simulink model "model8_train"  (R2024b)
settings: Solver=VariableStepAuto  StartTime=0.0  StopTime=24  RelTol=1e-3
model workspace (MAT data in the model file):
  agentObj = 67
undefined symbols (not defined in the file): bat_deseado, bat_inicial, difh, dni, e_inicial, ghi, glb, n_inicial, seed_radiation, seed_solar, seed_x, seed_y, seed_z, selection, sun_vector, viento
libraries: rllib x3
settings Model: Creator=danie  LastModifiedBy=Daniel
settings SolverCC: ZeroCrossAlgorithm=Adaptive
settings DebuggingCC: IgnoredZcDiagnostic=none

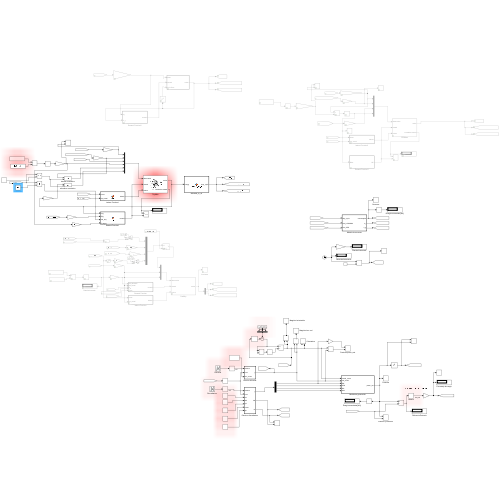
[thumbnail: Simulink's stored preview of the top-level diagram]
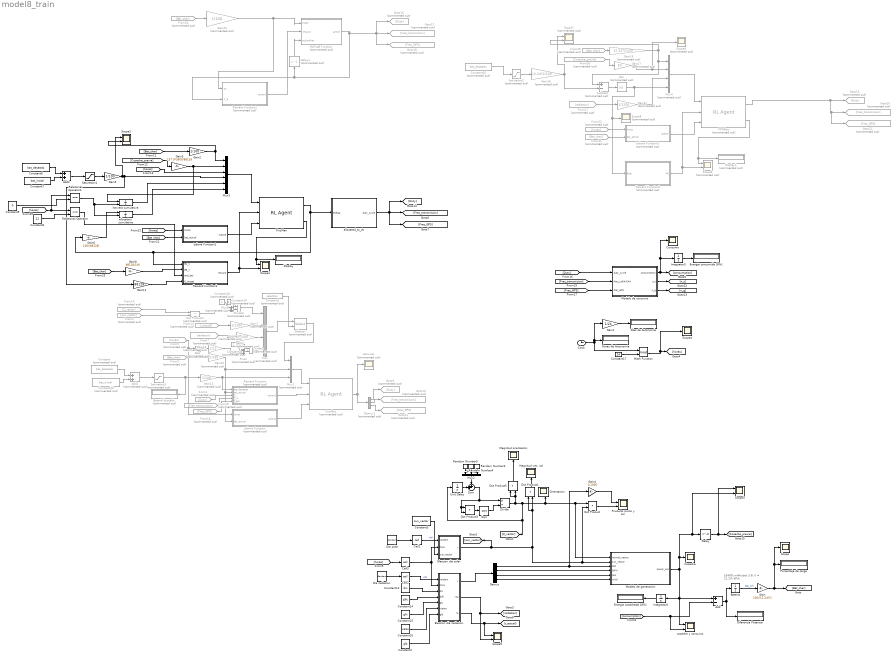
== system model8_train ==
  note: $3400\:mAh\cdot 3.6\:V = 12.24\:Wh$
  Abs : Abs  Commented=on  SaturateOnIntegerOverflow=off
  Acciones : Scope  Commented=on
  Add : Sum  Inputs=+-
  Add1 : Sum  Commented=on
  Add2 : Sum
  Batería : Integrator  InitialCondition=12.24*2*(bat_inicial/100)  LimitOutput=on  UpperSaturationLimit=12.24*2  LowerSaturationLimit=0
  Batería buscado : Display  Commented=on
  Bias : Bias  Commented=on  Bias=-12  SaturateOnIntegerOverflow=off
  Ceil1 : Rounding  Operator=ceil
  Ceil2 : Rounding  Operator=ceil
  Ceil3 : Rounding  Operator=ceil
  Clock : Clock
  Constant : Constant  Commented=on  Value=bat_deseado
  Constant1 : Constant  Commented=on  Value=selection
  Constant10 : Constant  Commented=on  Value=bat_deseado
  Constant13 : Constant  Value=dni
  Constant14 : Constant  Value=difh
  Constant15 : Constant  Value=ghi
  Constant16 : Constant  Value=viento
  Constant17 : Constant  Value=24
  Constant18 : Constant  Commented=on
  Constant19 : Constant  Commented=on  Value=2
  Constant2 : Constant  Value=glb
  Constant20 : Constant  Commented=on  Value=bat_inicial
  Constant3 : Constant  Value=sun_vector
  Constant4 : Constant  Commented=on
  Constant5 : Constant  Commented=on  Value=2
  Constant6 : Constant  Value=bat_deseado
  Constant7 : Constant  Value=bat_inicial
  Constant8 : Constant  Value=22
  Constant9 : Constant  Value=0
  Consumo : Scope
  Cosecha : Scope
  CowBoy : rllib/RL Agent  Commented=on  Agent=agent  ExternalActionAsInput=off  ProvideLastAction=off  ProvideCumRwd=off  TreatAsDirectFeedthrough=on  UseStrictObservationDataTypes=off
  Delay : Delay  DelayLength=0  SampleTime=1
  Delay1 : Delay  Commented=on  DelayLength=1
  Demux : Demux
  Demux1 : Demux  Commented=on  Outputs=3
  Diferencia Potencia : Display
  Display : Display
  Display1 : Display  Commented=on
  Divide : Product  Inputs=*/
  Divide1 : Product  Commented=on  Inputs=/*
  Divide3 : Product  Commented=on  Inputs=/*
  Dot Product{,1,3,5} (4 alike) : DotProduct  OutDataTypeStr=Inherit: Inherit via internal rule
  Dot Product4 : DotProduct  Commented=on  OutDataTypeStr=Inherit: Inherit via internal rule
  Día radiacion : UniformRandomNumber  Minimum=1  Maximum=4383  Seed=seed_radiation  SampleTime=24
  Día solar : UniformRandomNumber  Minimum=1  Maximum=365  Seed=seed_solar  SampleTime=24
  Días de Autonomía : Display
  Eleccion día radiacion : MATLAB Function  TreatAsAtomicUnit=on
  Eleccion día solar : MATLAB Function  TreatAsAtomicUnit=on
  Energia consumida [Wh] : Display
      settings: Decimation=5
  Energia cosechada [Wh] : Display
      settings: Decimation=5
  From1 : From  Commented=on  GotoTag=Duty
  From10 : From  Commented=on  GotoTag=Z_vector
  From14 : From  Commented=on  GotoTag=r_actual
  From18 : From  Commented=on  GotoTag=Frec_GPS
  From19 : From  Commented=on  GotoTag=Frec_transmision
  From2 : From  Commented=on  GotoTag=sun_vector
  From{3,24..25,31} (4 alike) : From  Commented=on  GotoTag=Bat_char
  From26 : From  Commented=on  GotoTag=Cosecha_previa
  From27 : From  Commented=on  GotoTag=radiation
  From32 : From  Commented=on  GotoTag=horas
  From5 : From  Commented=on  GotoTag=horas
  From7 : From  Commented=on  GotoTag=radiation
  Gain : Gain  Gain=100/(12.24*2)
  Gain1 : Gain  Gain=1/24
  Gain10 : Gain  Commented=on  Gain=1/100
  Gain11 : Gain  Gain=88128
  Gain12 : Gain  Commented=on  Gain=1/12
  Gain13 : Gain  Commented=on  Gain=1/100
  Gain15 : Gain  Commented=on  Gain=1/100
  Gain16 : Gain  Commented=on  Gain=12.24*2/100
  Gain17 : Gain  Commented=on  Gain=50
  Gain18 : Gain  Commented=on  Gain=12.24*2/100
  Gain2 : Gain  Gain=1/100
  Gain21 : Gain  Commented=on  Gain=1/1200
  Gain3 : Gain  Gain=157.5*3600/88128
  Gain4 : Gain  Gain=1/1000
  Gain5 : Gain  Gain=1/100
  Gain6 : Gain  Gain=100/(88128)
  Gain7 : Gain  Commented=on  Gain=1/1200
  Gain8 : Gain  Gain=88128/100
  Gain9 : Gain  Commented=on  Gain=1/1200
  Goto10 : Goto  Commented=on  GotoTag=Frec_transmision
  Goto11 : Goto  Commented=on  GotoTag=Frec_GPS
  Goto16 : Goto  Commented=on  GotoTag=Duty
  Goto17 : Goto  Commented=on  GotoTag=Frec_transmision
  Goto18 : Goto  Commented=on  GotoTag=Frec_GPS
  Goto19 : Goto  Commented=on  GotoTag=Duty
  Goto20 : Goto  Commented=on  GotoTag=Frec_transmision
  Goto21 : Goto  Commented=on  GotoTag=Frec_GPS
  Goto9 : Goto  Commented=on  GotoTag=Duty
  Horas de Autonomía : Display
  Integrator3 : Integrator
  Integrator6 : Integrator
  Isdone Function : MATLAB Function  Commented=on  TreatAsAtomicUnit=on
  Isdone Function1 : MATLAB Function  TreatAsAtomicUnit=on
  Isdone Function3 : MATLAB Function  Commented=on  TreatAsAtomicUnit=on
  MATLAB Function : MATLAB Function  Commented=on  TreatAsAtomicUnit=on
  Magnitud orientación : Scope
  Magnitud vec. sol : Scope
  Math Function : Math  Operator=mod
  Modelo de consumo : MATLAB Function  TreatAsAtomicUnit=on
  Modelo de generación : MATLAB Function  TreatAsAtomicUnit=on
  Mux : Mux  Commented=on
  Mux1 : Mux  Commented=on  Inputs=3
  Mux2 : Mux  Inputs=3
  Mux3 : Mux  Inputs=6
  Mux4 : Mux  Commented=on
  Orientacion : Scope  NumInputPorts=2
  PPOMan : rllib/RL Agent  Commented=on  Agent=agent  ExternalActionAsInput=off  ProvideLastAction=off  ProvideCumRwd=on  TreatAsDirectFeedthrough=on  UseStrictObservationDataTypes=off
  Plus1 : Sum  Commented=on
  Plus2 : Sum  Commented=on
  Porcentaje de carga : Display
  Producto punto y sol : Scope  NumInputPorts=2
  Random Number3 : RandomNumber  Variance=0.05  Seed=seed_x  SampleTime=1
  Random Number4 : RandomNumber  Variance=0.05  Seed=seed_y  SampleTime=1
  Random Number5 : RandomNumber  Variance=0.05  Seed=seed_z  SampleTime=1
  Relational Operator : RelationalOperator  OutDataTypeStr=boolean  ZeroCross=off  RndMeth=Simplest  InputSameDT=off
  Relational Operator1 : RelationalOperator  Operator===  OutDataTypeStr=boolean  ZeroCross=off  RndMeth=Simplest  InputSameDT=off
  Reward Function : MATLAB Function  Commented=on  TreatAsAtomicUnit=on
  Reward Function1 : MATLAB Function  TreatAsAtomicUnit=on
  Reward Function2 : MATLAB Function  Commented=on  TreatAsAtomicUnit=on
  Reward Function3 : MATLAB Function  Commented=on  TreatAsAtomicUnit=on
  Saturation1 : Saturate  UpperLimit=100  LowerLimit=1
  Saturation2 : Saturate  Commented=on  UpperLimit=100  LowerLimit=1
  Saturation3 : Saturate  Commented=on  UpperLimit=100  LowerLimit=1
  Scope : Scope
  Scope{1..3,5} (4 alike) : Scope  NumInputPorts=2
  Scope4 : Scope
  Scope6 : Scope  Commented=on  NumInputPorts=2
  Scope7 : Scope  Commented=on  NumInputPorts=2
  Scope8 : Scope  Commented=on
  Scope9 : Scope  Commented=on
  Selector : Selector  Commented=on  InputPortWidth=4  IndexOptions=Index vector (port)  Indices=[1 3]  OutputSizes=1
  Sqrt : Sqrt
  Subtract : Sum  Commented=on  Inputs=+-
  Sum : Sum  Inputs=++|
  TinyMan : rllib/RL Agent  Agent=agent  ExternalActionAsInput=off  ProvideLastAction=off  ProvideCumRwd=on  TreatAsDirectFeedthrough=on  UseStrictObservationDataTypes=off
  Unit Delay : UnitDelay  InitialCondition=[e_inicial n_inicial 1]  HasFrameUpgradeWarning=on
  allocated_to_dc : MATLAB Function  TreatAsAtomicUnit=on
  allocation cumulative : Integrator  ExternalReset=rising  UpperSaturationLimit=12.24*2  LowerSaturationLimit=0
  cosecha y consumo : Scope  NumInputPorts=2
  harvest cumulative : Integrator  ExternalReset=rising  UpperSaturationLimit=12.24*2  LowerSaturationLimit=0
  wires:
  Add/1 -> Batería/1, Diferencia Potencia/1
  Batería/1 -> Gain/1  "bat_wh"
  Gain/1 -> [Bat_char], Scope/1, Porcentaje de carga/1
  [consumption] -> cosecha y consumo/2, Add/2
  Clock/1 -> Math Function/1, Gain1/1, Horas de Autonomía/1
  Gain1/1 -> Días de Autonomía/1
  Demux/2 -> Modelo de generación/4(DIFH)
  Demux/3 -> Modelo de generación/5(GHI)
  Demux/4 -> Modelo de generación/6(wind)
  Eleccion día solar/1(y) -> Dot Product/2, Modelo de generación/2(sun_vector), Dot Product1/1, Dot Product1/2, [sun_vector]
  Dot Product/1 -> Producto punto y sol/2
  Dot Product1/1 -> Magnitud vec. sol/1
  Gain4/1 -> Producto punto y sol/1
  Mux/1 -> Selector/1
  Gain9/1 -> Mux/3
  From5/1 -> Isdone Function/1(horas), Bias/1
  Add1/1 -> Saturation3/1
  Sum/1 -> Dot Product3/2, Dot Product3/1, Divide/1
  Dot Product3/1 -> Sqrt/1
  Eleccion día radiacion/1(y) -> Demux/1
  Ceil3/1 -> Eleccion día radiacion/2(hora), Eleccion día solar/2(hora)
  Ceil1/1 -> Eleccion día solar/1(random)  "roll"
  Día solar/1 -> Ceil1/1
  Día radiacion/1 -> Ceil2/1
  Ceil2/1 -> Eleccion día radiacion/1(random)  "roll"
  Constant13/1 -> Eleccion día radiacion/3(dni)
  Constant14/1 -> Eleccion día radiacion/4(difh)
  Constant15/1 -> Eleccion día radiacion/5(ghi)
  Constant16/1 -> Eleccion día radiacion/6(viento)
  Constant3/1 -> Eleccion día solar/3(sun_vector)
  [horas] -> Ceil3/1
  From7/1 -> Gain9/1
  Gain10/1 -> Isdone Function/2(bat_actual), Reward Function/2(bat_actual), Mux1/2
  CowBoy/1 -> Demux1/1, Acciones/1
  Eleccion día radiacion/2(r24) -> [radiation], Scope5/2
  Bias/1 -> Gain12/1
  Modelo de consumo/1(consumption) -> Consumo/1, Integrator3/1, [consumption]
  Math Function/1 -> Scope4/1, [horas]
  Constant17/1 -> Math Function/2
  Gain13/1 -> Mux1/3, Reward Function/1(bat_deseado)
  Integrator3/1 -> Energia consumida [Wh]/1
  From3/1 -> Gain10/1
  Reward Function/1(reward) -> CowBoy/2
  Isdone Function/1(isdone) -> CowBoy/3
  From14/1 -> Gain7/1
  Gain7/1 -> Mux/2
  Constant/1 -> Add1/1
  Constant20/1 -> Add1/2
  Demux1/1 -> Goto9/1
  Demux1/2 -> Goto10/1
  Integrator6/1 -> Energia cosechada [Wh]/1
  Modelo de generación/1(power_out) -> Scope3/2, Delay/1, Cosecha/1, Add/1, cosecha y consumo/1, Integrator6/1
  Sqrt/1 -> Divide/2
  Dot Product5/1 -> Magnitud orientación/1
  Divide/1 -> Unit Delay/1, [Z_vector], Modelo de generación/1(normal_vector), Dot Product/1, Orientacion/2, Dot Product5/1, Dot Product5/2
  [Frec_transmision] -> Modelo de consumo/2(frec_LoRAWAN)
  [Frec_GPS] -> Modelo de consumo/3(frec_GPS)
  [Duty] -> Modelo de consumo/1(duty_cycle)
  Demux1/3 -> Goto11/1
  Modelo de consumo/2(n_t) -> [n_t]
  Modelo de consumo/3(n_g) -> [n_g]
  From19/1 -> Reward Function/4(f_tx)
  From18/1 -> Reward Function/5(f_gps)
  Unit Delay/1 -> Sum/2
  Random Number5/1 -> Mux2/3
  Random Number3/1 -> Mux2/1
  Random Number4/1 -> Mux2/2
  Mux2/1 -> Sum/1
  Eleccion día radiacion/3(ra) -> Scope5/1, [r_actual]
  Demux/1 -> Modelo de generación/3(DNI), Gain4/1
  Constant2/1 -> Eleccion día radiacion/7(glb)
  Mux1/1 -> CowBoy/1
  Selector/1 -> Mux1/1
  Constant1/1 -> Selector/2
  Constant18/1 -> Plus1/1
  Constant19/1 -> Divide3/1
  Plus1/1 -> Divide3/2
  Divide3/1 -> Mux/1
  Dot Product4/1 -> Plus1/2
  Constant4/1 -> Plus2/1
  Constant5/1 -> Divide1/1
  Plus2/1 -> Divide1/2
  Divide1/1 -> Mux/4
  Gain12/1 -> Plus2/2
  Saturation3/1 -> Batería buscado/1, Gain13/1
  From1/1 -> Reward Function/3(D)
  From10/1 -> Dot Product4/1
  From2/1 -> Dot Product4/2
  Isdone Function1/1(isdone) -> TinyMan/3
  Reward Function1/1(reward) -> Scope1/2, TinyMan/2
  Mux3/1 -> TinyMan/1
  allocated_to_dc/1(duty_cycle) -> [Frec_GPS], [Duty], [Frec_transmision]
  Delay/1 -> Scope3/1, [Cosecha_previa]
  [Bat_char] -> Gain2/1
  [Cosecha_previa] -> Gain3/1
  [horas] -> Mux3/3
  Constant7/1 -> Add2/2
  Add2/1 -> Saturation1/1
  Constant6/1 -> Add2/1
  Saturation1/1 -> Gain5/1
  Gain5/1 -> Scope2/1, Gain11/1, Mux3/4
  [horas] -> Relational Operator1/1, Relational Operator/1
  Constant8/1 -> Relational Operator/2
  Relational Operator/1 -> Reward Function1/3(end_day)
  harvest cumulative/1 -> Mux3/5
  [Bat_char] -> Isdone Function1/2(bat_actual)
  [horas] -> Isdone Function1/1(horas)
  TinyMan/1 -> Reward Function1/1(EA_t), Gain6/1, allocated_to_dc/1(energy)
  Gain6/1 -> allocation cumulative/1
  [Bat_char] -> Gain8/1
  Gain8/1 -> Reward Function1/2(EB_t)
  Gain11/1 -> Reward Function1/4(E_target)
  Reward Function2/1(reward) -> MATLAB Function/2(reward)
  From24/1 -> Gain15/1
  MATLAB Function/1(action) -> Goto18/1, Goto16/1, Goto17/1, Delay1/1, Reward Function2/2(X_g)
  Gain15/1 -> MATLAB Function/1(state), Reward Function2/1(e_r)
  Delay1/1 -> MATLAB Function/3(actionPrev)
  Gain2/1 -> Mux3/1, Scope2/2
  TinyMan/2 -> Display/1, Scope1/1
  allocation cumulative/1 -> Mux3/6
  Gain3/1 -> harvest cumulative/1, Mux3/2
  Constant9/1 -> Relational Operator1/2
  Relational Operator1/1 -> allocation cumulative/2, harvest cumulative/2
  From25/1 -> Gain16/1
  Isdone Function3/1(isdone) -> PPOMan/3
  Reward Function3/1(RE) -> Scope6/2, PPOMan/2
  From31/1 -> Isdone Function3/2(bat_actual)
  From32/1 -> Isdone Function3/1(horas)
  PPOMan/1 -> Goto21/1, Goto20/1, Goto19/1
  Constant10/1 -> Saturation2/1
  Gain17/1 -> Scope9/1, Mux4/2
  Gain16/1 -> Subtract/1, Mux4/1, Scope7/2
  Mux4/1 -> PPOMan/1
  Saturation2/1 -> Gain18/1
  PPOMan/2 -> Display1/1, Scope6/1
  From26/1 -> Gain17/1
  Subtract/1 -> Abs/1
  Abs/1 -> Scope8/1, Reward Function3/1(Edist), Mux4/4
  From27/1 -> Gain21/1
  Gain21/1 -> Mux4/3
  Gain18/1 -> Subtract/2, Scope7/1

== matlab function model8_train/allocated_to_dc ==
  data: energy input; duty_cycle output
function duty_cycle  = allocated_to_dc(energy)



duty_cycle = energy/112.715;

if (duty_cycle < 0.1)
    duty_cycle = 0.1;
end

if (duty_cycle > 1)
    duty_cycle = 1;
end


end

== matlab function model8_train/Reward Function2 ==
  data: e_r input; reward output; X_g input
function reward = fcn(e_r,X_g)

E_rmax = 1;
E_rfail = 0;

phi = (e_r-E_rfail)/(E_rmax-E_rfail);
reward = phi*x_g;

end

== matlab function model8_train/MATLAB Function ==
  data: state input; action output; reward input; actionPrev input
function action = RLAgent(state, reward, actionPrev)
% RLAgent: Implementación básica del algoritmo RLMan

% Parámetros globales del actor-crítico
persistent theta psi sigma gamma lambda alpha beta phiPrev value
if isempty(theta)
    % Inicialización de parámetros
    theta = 0; psi = 0; sigma = 0.1;
    gamma = 0.9; lambda = 0.9; alpha = 0.01; beta = 0.01;
    phiPrev = 0;
    value = 0;
end

action = 0;

% Normalizar el estado (energía residual)
E_fail = 0.1; % Energía mínima (modificar según configuración)
E_max = 1.0; % Energía máxima
phi = (state - E_fail) / (E_max - E_fail);

% Cálculo del error TD (Temporal Difference Error)
delta = reward + gamma * (theta * phi) - (theta * phiPrev);

% Actualización del Crítico (valor del estado)
value = gamma * lambda * value + phi
theta = theta + alpha * delta * value

% Actualización del Actor (parámetros de la política)
psi = psi + beta * delta * (actionPrev - (psi * phiPrev)) / sigma^2 * phiPrev;

% Política Gaussiana para seleccionar acción (tasa de paquetes)
mu = psi * phi;
action = mu + sigma * randn;

% Restricción de acción al rango permitido
X_min = 0.1; % Tasa mínima (modificar según configuración)
X_max = 1.0; % Tasa máxima
action = max(min(action, X_max), X_min);

% Actualizar estado previo
phiPrev = phi;
end

== matlab function model8_train/Isdone Function3 ==
  data: horas input; isdone output; bat_actual input
function isdone = fcn(horas,bat_actual)

    isdone = (horas==24)||(bat_actual<=0);

== matlab function model8_train/Reward Function3 ==
  data: Edist input; RE output
function RE = calcular_RE(Edist)

    if Edist < 0
        Edist = 0;
    end

    % Función para calcular RE basado en el valor de Edist
    if Edist == 0
        RE = 500;
    elseif Edist > 0 && Edist <= 1
        RE = 500 - Edist / 10;
    elseif Edist > 1 && Edist <= 5
        RE = 10 - Edist / 100;
    elseif Edist > 5
        RE = -500;
    else
        error('El valor de Edist no es válido');
    end
end

== matlab function model8_train/Modelo de generación ==
  data: normal_vector input; power_out output; sun_vector input; DNI input; DIFH input; GHI input; wind input
function power_out  = radiation_model(normal_vector,sun_vector,DNI,DIFH,GHI,wind)

%   By: Daniel Iglesias - UFRO - 2024

%   Modelo basado en "Modelo de Generación Fotovoltaica" de Alejandra
%   Molina Monje y Francisco martínez (Marzo 2017)
%   Disponible en: https://solar.minenergia.cl/downloads/fotovoltaico.pdf
%   [Consultado el 25-11-2024]

% Normal vector:
% Vector normal al panel solar, en formato:
% [Este, Norte, Zenith]
% 
% Sun vector:
% Vector de posición del sol, en formato:
% [Este, Norte, Zenith]

%% Parametros
efficiency = 0.34;
panel_power = 0.3; % Potencia nominal de la instalación
coef_temp = -0.002; % Coeficiencte de temperatura de la celda para su potencia máxima
I_o = 1000; % Radiación de referencia
T_o = 25; % Temperatura de referencia
dT = -0.0471;
a = -2.98;
b = -0.0471;
albedo = 0.24;

%% Módulo de Radiación

% Radiación directa:
dir_inc = max(0,DNI*dot(normal_vector,sun_vector));

% Radiación difusa del cielo
dif_inc = DIFH*0.5*(1 + dot(normal_vector,[0 0 1]));

% Radiación difusa del suelo
dif_suelo = GHI*0.5*albedo*(1 + dot(normal_vector,[0 0 1]));

% Radiación total que incide en un plano inclinado:
incident_rad = dir_inc + dif_inc + dif_suelo;

%% Módulo de reflexión

% El panel utilizado no presenta una cubierta, por lo que no se consideró
% el uso de este módulo.


%% Módulo de Temperatura

% Temperatura de celda:
T_c = dT*incident_rad/1000 + incident_rad*exp(a + b*wind);

%% Módulo de Operación

% Potencia generada
high_power = incident_rad/I_o*panel_power*(1 + coef_temp*(T_c-T_o));
low_power = 0.008*incident_rad^2/I_o * panel_power*(1 + coef_temp*(T_c-T_o));

if incident_rad >= 125
    power_generated = high_power;
else
    power_generated = low_power;
end

%% Módulo de Inversor & Módulo de Pérdidas

%power_out = efficiency*power_generated;
power_out = 1.4327*power_generated^3 - 1.5697*power_generated^2 + 0.6165*power_generated - 0.0005;

end

% glb [W/m2]: Radiación Global
% dir [W/m2]: Radiación Directa
% dif [W/m2]: Radiación Difusa
% sct [W/m2]: Radiación Difusa Relejada
% ghi [W/m2]: Radiación Global Horizontal
% dirh [W/m2]: Radiación Directa
% difh [W/m2]: Radiación Difusa
% dni [W/m2]: Radiación Directa Normal
% temp [C]: Temperatura en 2 metros (correjida)
% vel [m/s]: Velocidad de Viento
% shadow [0: sin, 1: con]: Sobra debido a topografía
% cloud [1: si, 0: no]: Presencia de nubes

== matlab function model8_train/Eleccion día solar ==
  data: random input; y output; hora input; sun_vector input
function y = fcn(random,hora,sun_vector)

y = zeros(3, 1);
hora = fix(hora);

n_inicial = (random-1)*24 + 1;

y(1) = sun_vector(n_inicial+hora,1);
y(2) = sun_vector(n_inicial+hora,2);
y(3) = sun_vector(n_inicial+hora,3);

== matlab function model8_train/Eleccion día radiacion ==
  data: random input; y output; hora input; dni input; difh input; ghi input; viento input; r24 output; ra output; glb input
function [y,r24,ra] = fcn(random,hora,dni,difh,ghi,viento,glb)

y = zeros(4, 1);
hora = fix(hora);
%r24 = zeros(24,1);

r24 = 0;

n_inicial = (random - 1)*24 + 1;
%n_final = n_inicial+24;

y(1) = dni(n_inicial+hora,2);
y(2) = difh(n_inicial+hora,2);
y(3) = ghi(n_inicial+hora,2);
y(4) = viento(n_inicial+hora,2);
ra = glb(n_inicial+hora,2);

for k = 0:23
    r24 = r24 + glb(n_inicial+k,2);
end

r24 = r24/24;


% y(1) = dni;
% y(2) = difh;
% y(3) = ghi;
% y(4) = viento;

== matlab function model8_train/Reward Function ==
  data: bat_deseado input; reward output; bat_actual input; D input; f_tx input; f_gps input
function reward = fcn(bat_deseado,bat_actual,D,f_tx,f_gps)

dif = abs(bat_deseado-bat_actual);

% 
% reward = 0.5*(dif<=0.02) - 0.05*dif - 10*(bat_actual<=0);

% %ORIGINAL:
% a=0.5;
% b=0.5;
% c=0.5;
% d=500;
% e=10;

a=10;
b=0.25;
c=0.25;
d=500;
e=10;


reward = a*D+b*f_tx+c*f_gps-d*dif-e*(bat_actual<=0);

== matlab function model8_train/Isdone Function ==
  data: horas input; isdone output; bat_actual input
function isdone = fcn(horas,bat_actual)

    isdone = (horas==24)||(bat_actual<=0);

== matlab function model8_train/Modelo de consumo ==
  data: duty_cycle input; consumption output; frec_LoRAWAN input; frec_GPS input; n_t output; n_g output
function [consumption,n_t,n_g] = consume_model(duty_cycle,frec_LoRAWAN, frec_GPS)


duty_cycle = min(max(duty_cycle, 0.1), 1);

%% Parametros
modo_activo = 0.095; % CPU
modo_lightsleep = 0.000792; % ULP
modo_deepsleep = 0.0000264; % Sleep

processing_time = 2/3600;

consumo_WT = 0.0000231;

icm42670_activo = 0.001814;
icm42670_sleep = 0.00001155;

transmision_power = 0.254;
transmision_time = 1.133/3600;

GPS_power = 0.437;
GPS_time = 48.520/3600;

%% Parametros JouleScope

modo_activo = 0; % CPU
modo_lightsleep = 0; % ULP
modo_deepsleep = 0; % Sleep

processing_time = 0;

consumo_WT = 0;

icm42670_activo = 0.00872307;
icm42670_sleep = 0.00156235;

%transmision_power = 0.17865;
transmision_power = 0.366;
transmision_time = 10.31/3600;

GPS_power = 0.49475;
GPS_time = 8.81/3600;

%% Ecuacion consumo

modo_activo_time = (duty_cycle*3600/10)*processing_time;
modo_deepsleep_time = 1 - modo_activo_time;

consumo_sensor = duty_cycle*icm42670_activo + (1-duty_cycle)*icm42670_sleep + modo_activo_time*modo_activo + modo_deepsleep_time*modo_deepsleep + consumo_WT;

if frec_LoRAWAN >= 1
    n_t = 10;
elseif frec_LoRAWAN >= 0.1
    n_t = fix(frec_LoRAWAN*10);
else
    n_t = 1;
end

if frec_GPS >= 1
    n_g = 10;
elseif frec_GPS >= 0.1
    n_g = fix(frec_GPS*10);
else
    n_g = 1;
end


consumo_gps = transmision_power*transmision_time*n_t;

consumo_transmision = GPS_power*GPS_time*n_g;

consumption = consumo_sensor + consumo_gps + consumo_transmision;

end

== matlab function model8_train/Isdone Function1 ==
  data: horas input; isdone output; bat_actual input
function isdone = fcn(horas,bat_actual)

    %isdone = (horas==24)||(bat_actual<=0);
    isdone = (horas==24);

== matlab function model8_train/Reward Function1 ==
  data: EA_t input; reward output; EB_t input; end_day input; E_target input
function reward = fcn(EA_t,EB_t,end_day,E_target)

reward = 0;

if end_day == false
    if EB_t >= 88128/100
        reward = log(EA_t/16.326);
    elseif EB_t < 88128/100 && EB_t > 0
        reward = -abs(EB_t-88128/100)/612;
    else
        reward = -abs(EB_t-E_target)/612;
    end

else 
    reward = -5*abs(EB_t-E_target)/612;
end
